simulink model "dairy_cip_digital_twin"  (R2026a)
settings: Solver=ode23t  StopTime=1900  MaxStep=5  RelTol=1e-4
PostLoadFcn:
  | try
  |     model_name = 'dairy_cip_digital_twin';
  |     model_file = get_param(model_name, 'FileName');
  |     if ~isempty(model_file)
  |         project_root = fileparts(fileparts(model_file));
  |     else
  |         project_root = pwd;
  |     end
  |     src_dir = fullfile(project_root, 'src');
  |     if ~isfolder(src_dir)
  |         src_dir = fullfile(pwd, 'src');
  |     end
  |     if isfolder(src_dir)
  |         addpath(src_dir);
  |     end
  | catch ME
  |     warning('dairy_cip_digital_twin:pathSetupFailed', ...
  |         'Could not add project src to MATLAB path: %s', ME.message);
  | end
InitFcn:
  | try
  |     model_name = 'dairy_cip_digital_twin';
  |     model_file = get_param(model_name, 'FileName');
  |     if ~isempty(model_file)
  |         project_root = fileparts(fileparts(model_file));
  |     else
  |         project_root = pwd;
  |     end
  |     src_dir = fullfile(project_root, 'src');
  |     if ~isfolder(src_dir)
  |         src_dir = fullfile(pwd, 'src');
  |     end
  |     if isfolder(src_dir)
  |         addpath(src_dir);
  |     end
  | catch ME
  |     warning('dairy_cip_digital_twin:pathSetupFailed', ...
  |         'Could not add project src to MATLAB path: %s', ME.message);
  | end
model workspace (MAT data in the model file):
  NaOH_pct = 1.5
  Q_m3h = 1.5
  T_C = 65
  T_in_C = 15
  heat_rec = 0.3
  soil0 = 0.6
  t_alk = 900
  t_final = 400
  t_int = 300
  t_pre = 300
  water_rec = 0.2
settings Model: Creator=OK  LastModifiedBy=OK

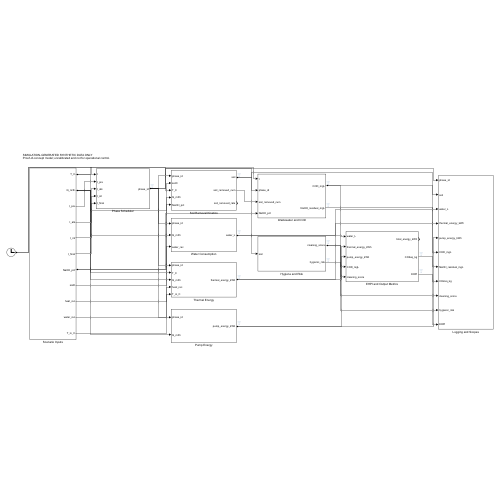
[thumbnail: Simulink's stored preview of the top-level diagram]
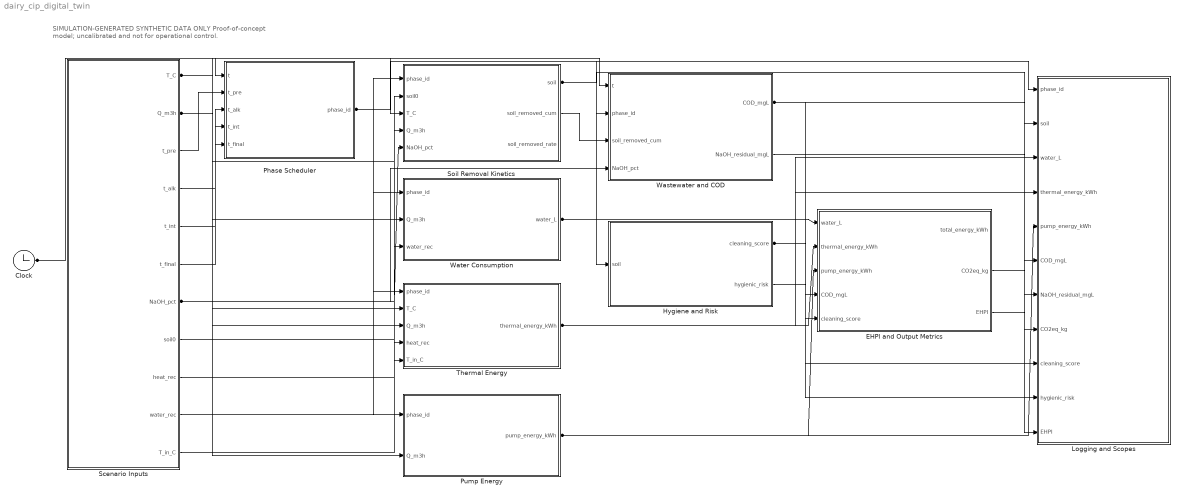
== system dairy_cip_digital_twin ==
  note: SIMULATION-GENERATED SYNTHETIC DATA ONLY
      | Proof-of-concept model; uncalibrated and not for operational control.
  Clock : Clock
  EHPI and Output Metrics : Subsystem
  Hygiene and Risk : Subsystem
  Logging and Scopes : Subsystem
  Phase Scheduler : Subsystem
  Pump Energy : Subsystem
  Scenario Inputs : Subsystem
  Soil Removal Kinetics : Subsystem
  Thermal Energy : Subsystem
  Wastewater and COD : Subsystem
  Water Consumption : Subsystem
  wires:
  Clock/1 -> Phase Scheduler/1(t), Wastewater and COD/1(t)
  Scenario Inputs/3(t_pre) -> Phase Scheduler/2(t_pre)
  Scenario Inputs/4(t_alk) -> Phase Scheduler/3(t_alk)
  Scenario Inputs/5(t_int) -> Phase Scheduler/4(t_int)
  Scenario Inputs/6(t_final) -> Phase Scheduler/5(t_final)
  Phase Scheduler/1(phase_id) -> Soil Removal Kinetics/1(phase_id), Water Consumption/1(phase_id), Thermal Energy/1(phase_id), Pump Energy/1(phase_id), Wastewater and COD/2(phase_id), Logging and Scopes/1(phase_id)
  Scenario Inputs/8(soil0) -> Soil Removal Kinetics/2(soil0)
  Scenario Inputs/1(T_C) -> Soil Removal Kinetics/3(T_C), Thermal Energy/2(T_C)
  Scenario Inputs/2(Q_m3h) -> Soil Removal Kinetics/4(Q_m3h), Water Consumption/2(Q_m3h), Thermal Energy/3(Q_m3h), Pump Energy/2(Q_m3h)
  Scenario Inputs/7(NaOH_pct) -> Soil Removal Kinetics/5(NaOH_pct), Wastewater and COD/4(NaOH_pct)
  Scenario Inputs/10(water_rec) -> Water Consumption/3(water_rec)
  Scenario Inputs/9(heat_rec) -> Thermal Energy/4(heat_rec)
  Scenario Inputs/11(T_in_C) -> Thermal Energy/5(T_in_C)
  Soil Removal Kinetics/2(soil_removed_cum) -> Wastewater and COD/3(soil_removed_cum)
  Soil Removal Kinetics/1(soil) -> Hygiene and Risk/1(soil), Logging and Scopes/2(soil)
  Water Consumption/1(water_L) -> EHPI and Output Metrics/1(water_L), Logging and Scopes/3(water_L)
  Thermal Energy/1(thermal_energy_kWh) -> EHPI and Output Metrics/2(thermal_energy_kWh), Logging and Scopes/4(thermal_energy_kWh)
  Pump Energy/1(pump_energy_kWh) -> EHPI and Output Metrics/3(pump_energy_kWh), Logging and Scopes/5(pump_energy_kWh)
  Wastewater and COD/1(COD_mgL) -> EHPI and Output Metrics/4(COD_mgL), Logging and Scopes/6(COD_mgL)
  Hygiene and Risk/1(cleaning_score) -> EHPI and Output Metrics/5(cleaning_score), Logging and Scopes/9(cleaning_score)
  Wastewater and COD/2(NaOH_residual_mgL) -> Logging and Scopes/7(NaOH_residual_mgL)
  EHPI and Output Metrics/2(CO2eq_kg) -> Logging and Scopes/8(CO2eq_kg)
  Hygiene and Risk/2(hygienic_risk) -> Logging and Scopes/10(hygienic_risk)
  EHPI and Output Metrics/3(EHPI) -> Logging and Scopes/11(EHPI)

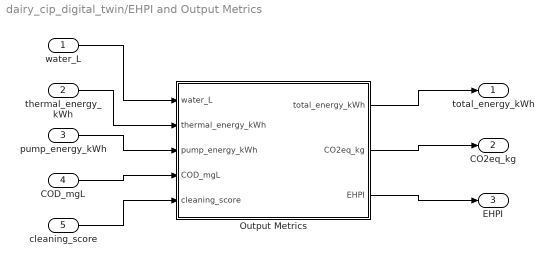
== system dairy_cip_digital_twin/EHPI and Output Metrics ==
  water_L : Inport
  thermal_energy_kWh : Inport  Port=2
  pump_energy_kWh : Inport  Port=3
  COD_mgL : Inport  Port=4
  cleaning_score : Inport  Port=5
  Output Metrics : MATLAB Function  TreatAsAtomicUnit=on
  total_energy_kWh : Outport
  CO2eq_kg : Outport  Port=2
  EHPI : Outport  Port=3
  wires:
  water_L/1 -> Output Metrics/1(water_L)
  thermal_energy_kWh/1 -> Output Metrics/2(thermal_energy_kWh)
  pump_energy_kWh/1 -> Output Metrics/3(pump_energy_kWh)
  COD_mgL/1 -> Output Metrics/4(COD_mgL)
  cleaning_score/1 -> Output Metrics/5(cleaning_score)
  Output Metrics/1(total_energy_kWh) -> total_energy_kWh/1
  Output Metrics/2(CO2eq_kg) -> CO2eq_kg/1
  Output Metrics/3(EHPI) -> EHPI/1

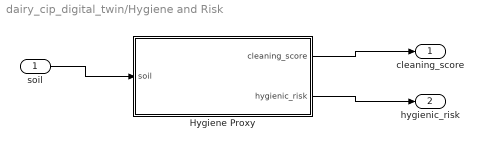
== system dairy_cip_digital_twin/Hygiene and Risk ==
  soil : Inport
  Hygiene Proxy : MATLAB Function  TreatAsAtomicUnit=on
  cleaning_score : Outport
  hygienic_risk : Outport  Port=2
  wires:
  soil/1 -> Hygiene Proxy/1(soil)
  Hygiene Proxy/1(cleaning_score) -> cleaning_score/1
  Hygiene Proxy/2(hygienic_risk) -> hygienic_risk/1

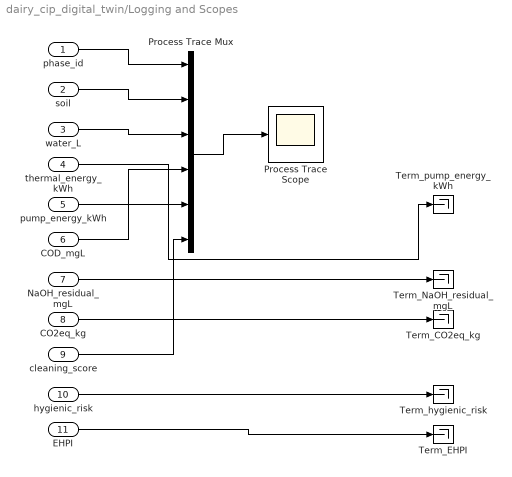
== system dairy_cip_digital_twin/Logging and Scopes ==
  phase_id : Inport
  soil : Inport  Port=2
  water_L : Inport  Port=3
  thermal_energy_kWh : Inport  Port=4
  pump_energy_kWh : Inport  Port=5
  COD_mgL : Inport  Port=6
  NaOH_residual_mgL : Inport  Port=7
  CO2eq_kg : Inport  Port=8
  cleaning_score : Inport  Port=9
  hygienic_risk : Inport  Port=10
  EHPI : Inport  Port=11
  Process Trace Mux : Mux  Inputs=6
  Process Trace Scope : Scope
  Term_CO2eq_kg : Terminator
  Term_EHPI : Terminator
  Term_NaOH_residual_mgL : Terminator
  Term_hygienic_risk : Terminator
  Term_pump_energy_kWh : Terminator
  wires:
  phase_id/1 -> Process Trace Mux/1
  soil/1 -> Process Trace Mux/2
  water_L/1 -> Process Trace Mux/3
  COD_mgL/1 -> Process Trace Mux/4
  thermal_energy_kWh/1 -> Process Trace Mux/5
  cleaning_score/1 -> Process Trace Mux/6
  Process Trace Mux/1 -> Process Trace Scope/1
  pump_energy_kWh/1 -> Term_pump_energy_kWh/1
  NaOH_residual_mgL/1 -> Term_NaOH_residual_mgL/1
  CO2eq_kg/1 -> Term_CO2eq_kg/1
  hygienic_risk/1 -> Term_hygienic_risk/1
  EHPI/1 -> Term_EHPI/1

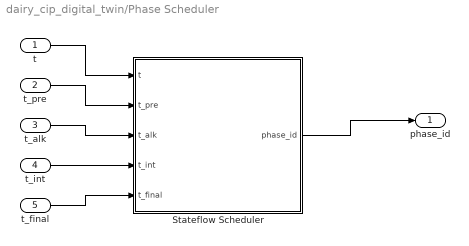
== system dairy_cip_digital_twin/Phase Scheduler ==
  t : Inport
  t_pre : Inport  Port=2
  t_alk : Inport  Port=3
  t_int : Inport  Port=4
  t_final : Inport  Port=5
  Stateflow Scheduler : Stateflow chart  TreatAsAtomicUnit=on
  phase_id : Outport
  wires:
  t/1 -> Stateflow Scheduler/1(t)
  t_pre/1 -> Stateflow Scheduler/2(t_pre)
  t_alk/1 -> Stateflow Scheduler/3(t_alk)
  t_int/1 -> Stateflow Scheduler/4(t_int)
  t_final/1 -> Stateflow Scheduler/5(t_final)
  Stateflow Scheduler/1(phase_id) -> phase_id/1

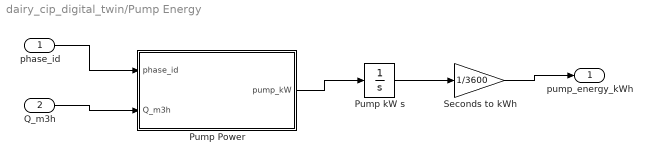
== system dairy_cip_digital_twin/Pump Energy ==
  phase_id : Inport
  Q_m3h : Inport  Port=2
  Pump Power : MATLAB Function  TreatAsAtomicUnit=on
  Pump kW s : Integrator
  Seconds to kWh : Gain  Gain=1/3600
  pump_energy_kWh : Outport
  wires:
  phase_id/1 -> Pump Power/1(phase_id)
  Q_m3h/1 -> Pump Power/2(Q_m3h)
  Pump Power/1(pump_kW) -> Pump kW s/1
  Pump kW s/1 -> Seconds to kWh/1
  Seconds to kWh/1 -> pump_energy_kWh/1

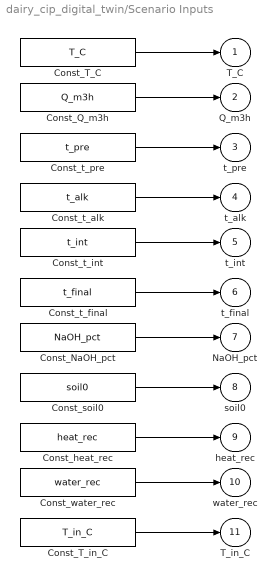
== system dairy_cip_digital_twin/Scenario Inputs ==
  Const_NaOH_pct : Constant  Value=NaOH_pct
  Const_Q_m3h : Constant  Value=Q_m3h
  Const_T_C : Constant  Value=T_C
  Const_T_in_C : Constant  Value=T_in_C
  Const_heat_rec : Constant  Value=heat_rec
  Const_soil0 : Constant  Value=soil0
  Const_t_alk : Constant  Value=t_alk
  Const_t_final : Constant  Value=t_final
  Const_t_int : Constant  Value=t_int
  Const_t_pre : Constant  Value=t_pre
  Const_water_rec : Constant  Value=water_rec
  T_C : Outport
  Q_m3h : Outport  Port=2
  t_pre : Outport  Port=3
  t_alk : Outport  Port=4
  t_int : Outport  Port=5
  t_final : Outport  Port=6
  NaOH_pct : Outport  Port=7
  soil0 : Outport  Port=8
  heat_rec : Outport  Port=9
  water_rec : Outport  Port=10
  T_in_C : Outport  Port=11
  wires:
  Const_T_C/1 -> T_C/1
  Const_Q_m3h/1 -> Q_m3h/1
  Const_t_pre/1 -> t_pre/1
  Const_t_alk/1 -> t_alk/1
  Const_t_int/1 -> t_int/1
  Const_t_final/1 -> t_final/1
  Const_NaOH_pct/1 -> NaOH_pct/1
  Const_soil0/1 -> soil0/1
  Const_heat_rec/1 -> heat_rec/1
  Const_water_rec/1 -> water_rec/1
  Const_T_in_C/1 -> T_in_C/1

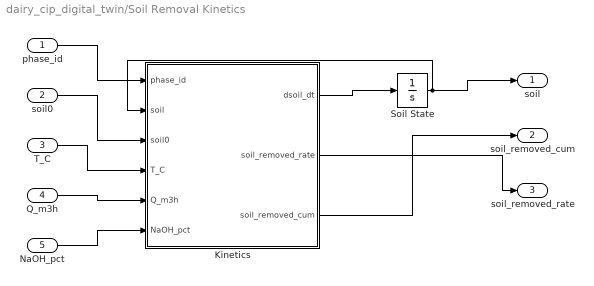
== system dairy_cip_digital_twin/Soil Removal Kinetics ==
  phase_id : Inport
  soil0 : Inport  Port=2
  T_C : Inport  Port=3
  Q_m3h : Inport  Port=4
  NaOH_pct : Inport  Port=5
  Kinetics : MATLAB Function  TreatAsAtomicUnit=on
  Soil State : Integrator  InitialCondition=soil0
  soil : Outport
  soil_removed_cum : Outport  Port=2
  soil_removed_rate : Outport  Port=3
  wires:
  phase_id/1 -> Kinetics/1(phase_id)
  Soil State/1 -> Kinetics/2(soil), soil/1
  soil0/1 -> Kinetics/3(soil0)
  T_C/1 -> Kinetics/4(T_C)
  Q_m3h/1 -> Kinetics/5(Q_m3h)
  NaOH_pct/1 -> Kinetics/6(NaOH_pct)
  Kinetics/1(dsoil_dt) -> Soil State/1
  Kinetics/3(soil_removed_cum) -> soil_removed_cum/1
  Kinetics/2(soil_removed_rate) -> soil_removed_rate/1

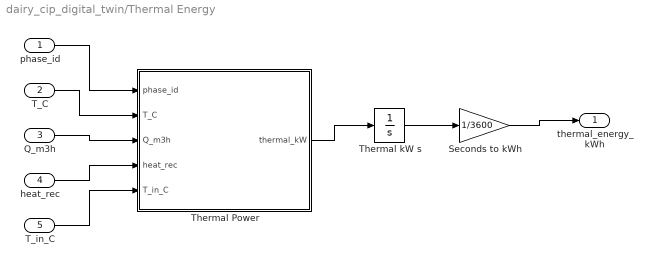
== system dairy_cip_digital_twin/Thermal Energy ==
  phase_id : Inport
  T_C : Inport  Port=2
  Q_m3h : Inport  Port=3
  heat_rec : Inport  Port=4
  T_in_C : Inport  Port=5
  Seconds to kWh : Gain  Gain=1/3600
  Thermal Power : MATLAB Function  TreatAsAtomicUnit=on
  Thermal kW s : Integrator
  thermal_energy_kWh : Outport
  wires:
  phase_id/1 -> Thermal Power/1(phase_id)
  T_C/1 -> Thermal Power/2(T_C)
  Q_m3h/1 -> Thermal Power/3(Q_m3h)
  heat_rec/1 -> Thermal Power/4(heat_rec)
  T_in_C/1 -> Thermal Power/5(T_in_C)
  Thermal Power/1(thermal_kW) -> Thermal kW s/1
  Thermal kW s/1 -> Seconds to kWh/1
  Seconds to kWh/1 -> thermal_energy_kWh/1

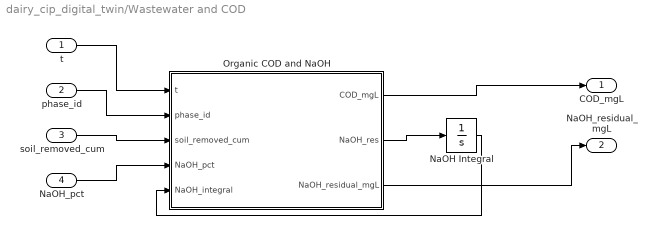
== system dairy_cip_digital_twin/Wastewater and COD ==
  t : Inport
  phase_id : Inport  Port=2
  soil_removed_cum : Inport  Port=3
  NaOH_pct : Inport  Port=4
  NaOH Integral : Integrator
  Organic COD and NaOH : MATLAB Function  TreatAsAtomicUnit=on
  COD_mgL : Outport
  NaOH_residual_mgL : Outport  Port=2
  wires:
  t/1 -> Organic COD and NaOH/1(t)
  phase_id/1 -> Organic COD and NaOH/2(phase_id)
  soil_removed_cum/1 -> Organic COD and NaOH/3(soil_removed_cum)
  NaOH_pct/1 -> Organic COD and NaOH/4(NaOH_pct)
  NaOH Integral/1 -> Organic COD and NaOH/5(NaOH_integral)
  Organic COD and NaOH/1(COD_mgL) -> COD_mgL/1
  Organic COD and NaOH/2(NaOH_res) -> NaOH Integral/1
  Organic COD and NaOH/3(NaOH_residual_mgL) -> NaOH_residual_mgL/1

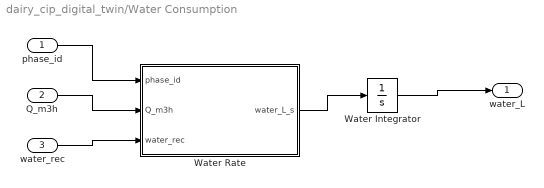
== system dairy_cip_digital_twin/Water Consumption ==
  phase_id : Inport
  Q_m3h : Inport  Port=2
  water_rec : Inport  Port=3
  Water Integrator : Integrator
  Water Rate : MATLAB Function  TreatAsAtomicUnit=on
  water_L : Outport
  wires:
  phase_id/1 -> Water Rate/1(phase_id)
  Q_m3h/1 -> Water Rate/2(Q_m3h)
  water_rec/1 -> Water Rate/3(water_rec)
  Water Rate/1(water_L_s) -> Water Integrator/1
  Water Integrator/1 -> water_L/1

== matlab function dairy_cip_digital_twin/Water Consumption/Water Rate ==
  data: phase_id input; water_L_s output; Q_m3h input; water_rec input
function water_L_s = water_rate(phase_id, Q_m3h, water_rec) %#codegen
%WATER_RATE Fresh-water flow during active CIP phases.
if phase_id >= 1 && phase_id <= 4
    water_L_s = Q_m3h * 1000 / 3600 * (1 - water_rec);
else
    water_L_s = 0;
end
end

== matlab function dairy_cip_digital_twin/Soil Removal Kinetics/Kinetics ==
  data: phase_id input; dsoil_dt output; soil input; soil0 input; T_C input; Q_m3h input; NaOH_pct input; soil_removed_rate output; soil_removed_cum output
function [dsoil_dt, soil_removed_rate, soil_removed_cum] = kinetics(phase_id, soil, soil0, T_C, Q_m3h, NaOH_pct) %#codegen
%KINETICS First-order soil removal for synthetic dairy CIP.
M = cip_model_params();
soil_c = max(soil, 0);
if phase_id == 1
    k = M.k_cal * M.k_pre_base * (Q_m3h / M.Q_ref)^M.beta_Q;
elseif phase_id == 2
    k = M.k_cal * M.k_alk_base * exp(M.alpha_T*(T_C - M.T_ref)) * ...
        (Q_m3h / M.Q_ref)^M.beta_Q * (NaOH_pct / M.NaOH_ref)^M.gamma_NaOH;
elseif phase_id == 3 || phase_id == 4
    k = M.k_cal * M.k_rinse_base * (Q_m3h / M.Q_ref)^M.beta_Q;
else
    k = 0;
end
dsoil_dt = -k * soil_c;
soil_removed_rate = max(-dsoil_dt, 0);
soil_removed_cum = min(max(soil0 - soil_c, 0), max(soil0, 0));
end

== stateflow chart dairy_cip_digital_twin/Phase Scheduler/Stateflow Scheduler ==
  state PRE_RINSE
    entry: phase_id = 1;
  state ALKALINE_WASH
    entry: phase_id = 2;
  state INTERMEDIATE_RINSE
    entry: phase_id = 3;
  state FINAL_RINSE
    entry: phase_id = 4;
  state ENDING
    entry: phase_id = 5;
  (default) -> PRE_RINSE
  PRE_RINSE -> ALKALINE_WASH : [t > t_pre]
  ALKALINE_WASH -> INTERMEDIATE_RINSE : [t > t_pre + t_alk]
  INTERMEDIATE_RINSE -> FINAL_RINSE : [t > t_pre + t_alk + t_int]
  FINAL_RINSE -> ENDING : [t > t_pre + t_alk + t_int + t_final]
  data: t input; t_pre input; t_alk input; t_int input; t_final input; phase_id output

== matlab function dairy_cip_digital_twin/Thermal Energy/Thermal Power ==
  data: phase_id input; thermal_kW output; T_C input; Q_m3h input; heat_rec input; T_in_C input
function thermal_kW = thermal_power(phase_id, T_C, Q_m3h, heat_rec, T_in_C) %#codegen
%THERMAL_POWER Heating power for the alkaline wash phase.
M = cip_model_params();
if phase_id == 2
    Q_m3s = Q_m3h / 3600;
    m_dot = M.rho * Q_m3s;
    dTemp = max(T_C - T_in_C, 0);
    thermal_kW = m_dot * M.cp * dTemp / M.eta_heater * (1 - heat_rec);
else
    thermal_kW = 0;
end
end

== matlab function dairy_cip_digital_twin/Pump Energy/Pump Power ==
  data: phase_id input; pump_kW output; Q_m3h input
function pump_kW = pump_power(phase_id, Q_m3h) %#codegen
%PUMP_POWER Pumping power during active CIP phases.
M = cip_model_params();
if phase_id >= 1 && phase_id <= 4
    Q_m3s = Q_m3h / 3600;
    pump_kW = (M.deltaP * Q_m3s / M.eta_pump) / 1000;
else
    pump_kW = 0;
end
end

== matlab function dairy_cip_digital_twin/Wastewater and COD/Organic COD and NaOH ==
  data: t input; COD_mgL output; phase_id input; soil_removed_cum input; NaOH_pct input; NaOH_integral input; NaOH_res output; NaOH_residual_mgL output
function [COD_mgL, NaOH_res, NaOH_residual_mgL] = wastewater_cod(t, phase_id, soil_removed_cum, NaOH_pct, NaOH_integral) %#codegen
%WASTEWATER_COD Organic COD proxy and separate NaOH residual reporting.
M = cip_model_params();
COD_mgL = M.COD_factor * max(soil_removed_cum, 0);
if phase_id == 2
    NaOH_res = NaOH_pct * 10000;
elseif phase_id == 3
    NaOH_res = NaOH_pct * 1500;
elseif phase_id == 4
    NaOH_res = NaOH_pct * 300;
else
    NaOH_res = 0;
end
NaOH_residual_mgL = NaOH_integral / max(t, M.eps_time);
end

== matlab function dairy_cip_digital_twin/Hygiene and Risk/Hygiene Proxy ==
  data: soil input; cleaning_score output; hygienic_risk output
function [cleaning_score, hygienic_risk] = hygiene_proxy(soil) %#codegen
%HYGIENE_PROXY Residual-soil hygiene proxies for synthetic data.
M = cip_model_params();
soil_c = max(soil, 0);
cleaning_score = max(0, min(100, (1 - soil_c) * 100));
hygienic_risk = max(0, min(1, soil_c / M.soil_risk_ref));
end

== matlab function dairy_cip_digital_twin/EHPI and Output Metrics/Output Metrics ==
  data: water_L input; total_energy_kWh output; thermal_energy_kWh input; pump_energy_kWh input; COD_mgL input; cleaning_score input; CO2eq_kg output; EHPI output
function [total_energy_kWh, CO2eq_kg, EHPI] = output_metrics(water_L, thermal_energy_kWh, pump_energy_kWh, COD_mgL, cleaning_score) %#codegen
%OUTPUT_METRICS Derived synthetic environmental and hygiene metrics.
M = cip_model_params();
total_energy_kWh = thermal_energy_kWh + pump_energy_kWh;
CO2eq_kg = thermal_energy_kWh * M.EF_thermal + pump_energy_kWh * M.EF_electricity;
water_norm = water_L / M.norm_water_L;
energy_norm = total_energy_kWh / M.norm_energy_kWh;
COD_norm = COD_mgL / M.norm_COD_mgL;
CO2_norm = CO2eq_kg / M.norm_CO2eq_kg;
cleaning_norm = cleaning_score / 100;
penalty_env = 0.25*water_norm + 0.25*energy_norm + 0.25*COD_norm + 0.25*CO2_norm;
EHPI = 100 * cleaning_norm / (1 + penalty_env);
end
